simulink model "cartpole"  (R2026a)
settings: Solver=VariableStepAuto  StopTime=20
values from neighbouring files (symbols this model uses):
  Fmax = 20    [setup_cartpole.m]
  K_lqr = dlqr(Ad,Bd,Q_lqr,R_lqr)    [setup_cartpole.m]
  m = model.m    [setup_cartpole.m]
  N = numel(U)    [backward_lqr.m]    (also in forward_pass.m; ilqr.m = numel(U0); linearize_trajectory.m; setup_cartpole.m = round(T/Ts))
  s = Q*xbar          + Ak'*snext          + Ak'*Snext*Bk*d(k)    [backward_lqr.m]
  Ts = 0.01    [setup_cartpole.m]
  X = Xnew    [ilqr.m]
undefined symbols (not defined in the file or in its folder): Knom, param, Unom, Xnom, Y, Z
libraries: sm_lib x11, nesl_utility x7
settings Model: Creator=basak  LastModifiedBy=paolapinna
settings SimscapeCC: SimscapeNominalValues="[{\"value\":\"1\",\"unit\":\"A\"},{\"value\":\"1\",\"unit\":\"bar\"},{\"value\":\"1\",\"unit\":\"cm^2\"},{\"value\":\"1\",\"unit\":\"cm^3/s\"},{\"value\":\"1\",\"unit\":\"kJ/kg\"},{\"value\":\"1\",\"unit\":\"kW\"},{\"value\":\"1\",\"unit\":\"l\"},{\"value\":\"1\",\"unit\":\"N\"},{\"value\":\"1\",\"unit\":\"N*m\"},{\"value\":\"1\",\"unit\":\"V\"}]"  SimscapeLogType=none  SimscapeLogDataHistory=5000.0

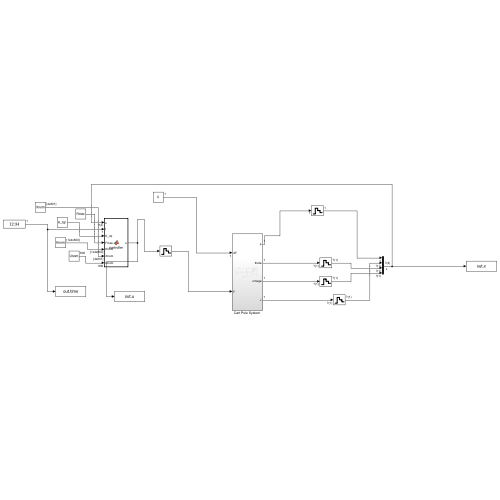
[thumbnail: Simulink's stored preview of the top-level diagram]
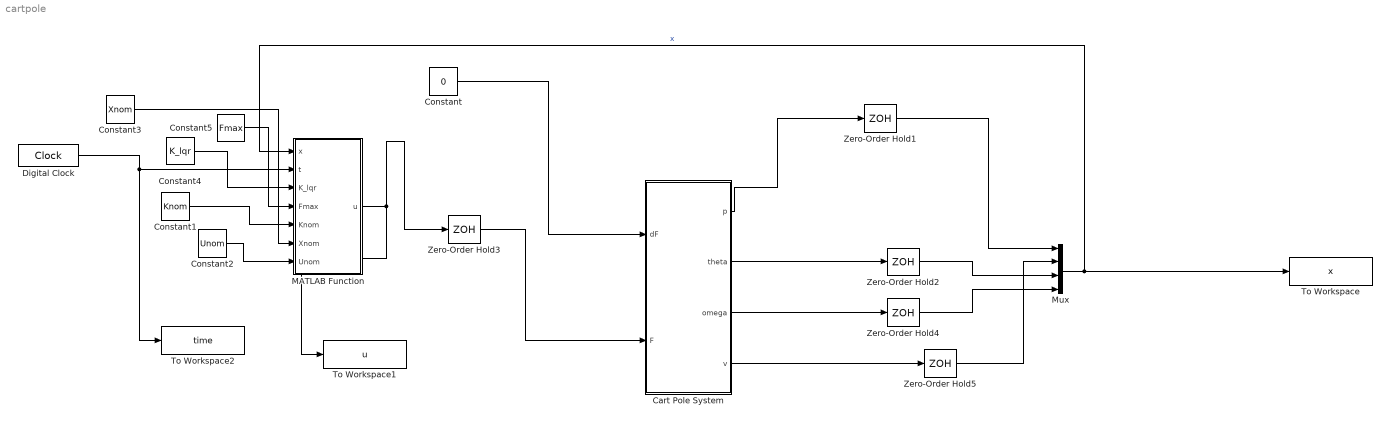
== system cartpole ==
  "Cart Pole System " : Subsystem
  Constant : Constant  Value=0
  Constant1 : Constant  Value=Knom
  Constant2 : Constant  Value=Unom
  Constant3 : Constant  Value=Xnom
  Constant4 : Constant  Value=K_lqr
  Constant5 : Constant  Value=Fmax
  Digital Clock : DigitalClock  SampleTime=Ts
  MATLAB Function : MATLAB Function  TreatAsAtomicUnit=on
  Mux : Mux
  To Workspace : ToWorkspace  VariableName=x  SaveFormat=Timeseries  SampleTime=-1
  To Workspace1 : ToWorkspace  VariableName=u  SaveFormat=Timeseries  SampleTime=-1
  To Workspace2 : ToWorkspace  VariableName=time  SaveFormat=Timeseries  SampleTime=-1
  Zero-Order Hold{1..5} (5 alike) : ZeroOrderHold  SampleTime=Ts
  wires:
  Constant/1 -> "Cart Pole System "/1(dF)
  "Cart Pole System "/1(p) -> Zero-Order Hold1/1
  "Cart Pole System "/2(theta) -> Zero-Order Hold2/1
  "Cart Pole System "/3(omega) -> Zero-Order Hold4/1
  "Cart Pole System "/4(v) -> Zero-Order Hold5/1
  MATLAB Function/1(u) -> Zero-Order Hold3/1, To Workspace1/1
  Zero-Order Hold3/1 -> "Cart Pole System "/2(F)
  Zero-Order Hold1/1 -> Mux/1
  Zero-Order Hold2/1 -> Mux/3
  Zero-Order Hold5/1 -> Mux/2
  Zero-Order Hold4/1 -> Mux/4
  Mux/1 -> To Workspace/1, MATLAB Function/1(x)  "x"
  Digital Clock/1 -> To Workspace2/1, MATLAB Function/2(t)
  Constant3/1 -> MATLAB Function/6(Xnom)
  Constant1/1 -> MATLAB Function/5(Knom)
  Constant2/1 -> MATLAB Function/7(Unom)
  Constant4/1 -> MATLAB Function/3(K_lqr)
  Constant5/1 -> MATLAB Function/4(Fmax)

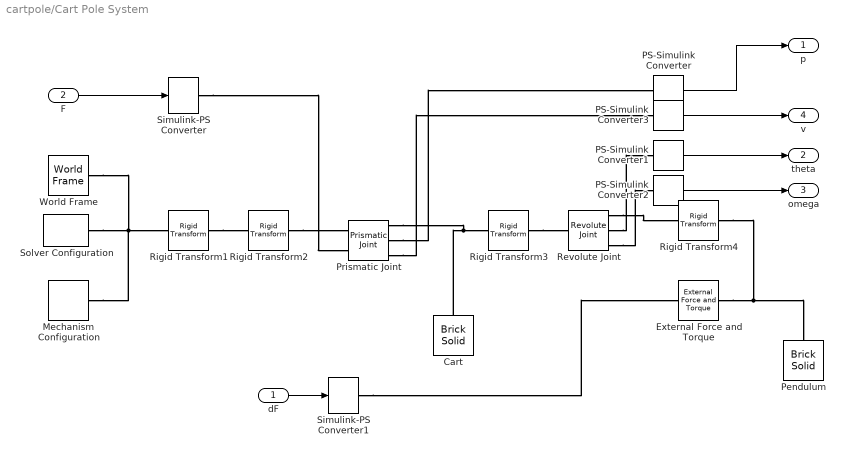
== system cartpole/Cart Pole System  ==
  dF : Inport
  F : Inport  Port=2
  Cart : sm_lib/Body Elements/Brick Solid  BrickDimensions=[param.L/6 param.L/6 param.L/3]  BrickDimensionsUnits=m  ExportEntireGeometry=off  InertiaType=PointMass  BasedOnType=Density  Density=1000  DensityUnits=kg/(m^3)  Mass=param.M  MassUnits=kg  CenterOfMass=[0 0 0]  CenterOfMassUnits=m  MomentsOfInertia=[1 1 1]  MomentsOfInertiaUnits=kg*m^2  ProductsOfInertia=[0 0 0]  ProductsOfInertiaUnits=kg*m^2  GraphicType=FromGeometry  MarkerShape=Sphere  MarkerSize=10  GraphicVisPropType=SimpleVisualProperties  GraphicDiffuseColor=[0.5 0.5 0.5]  GraphicOpacity=1.0  GraphicSpecularColor=[0.5 0.5 0.5 1.0]  GraphicAmbientColor=[0.15 0.15 0.15 1.0]  GraphicEmissiveColor=[0.0 0.0 0.0 1.0]  GraphicShininess=75  DoExposeReferenceFrame=on  SerializedFrames=<Frames/>
  External Force and Torque : sm_lib/Forces and Torques/External Force and Torque  EnableForceX=on  EnableForceY=off  EnableForceZ=off  EnableForce=off  ForceResolutionFrame=World  EnableTorqueX=off  EnableTorqueY=off  EnableTorqueZ=off  EnableTorque=off  TorqueResolutionFrame=AttachedFrame
  Mechanism Configuration : sm_lib/Utilities/Mechanism Configuration  UniformGravity=Constant  GravityVector=[0 0 -9.81]  GravityVectorUnits=m/s^2  LinearizationDelta=0.001  JointModeTransitionNonlinearIterations=2
  PS-Simulink Converter{,1..3} (4 alike) : nesl_utility/PS-Simulink Converter  PhysicalDomain=network_engine_domain  SubClassName=ps_output  LeftPortType=input  RightPortType=output  PseudoPeriodic=off  Frequencies=[]  VectorFormat=1-D array  Unit=1  AffineConversion=off
  Pendulum : sm_lib/Body Elements/Brick Solid  BrickDimensions=[param.L param.L/12 param.L/12]  BrickDimensionsUnits=m  ExportEntireGeometry=off  InertiaType=PointMass  BasedOnType=Density  Density=1000  DensityUnits=kg/(m^3)  Mass=param.m  MassUnits=kg  CenterOfMass=[0 0 0]  CenterOfMassUnits=m  MomentsOfInertia=[1 1 1]  MomentsOfInertiaUnits=kg*m^2  ProductsOfInertia=[0 0 0]  ProductsOfInertiaUnits=kg*m^2  GraphicType=FromGeometry  MarkerShape=Sphere  MarkerSize=10  GraphicVisPropType=SimpleVisualProperties  GraphicDiffuseColor=[0.8 0.0 0.2]  GraphicOpacity=1.0  GraphicSpecularColor=[0.5 0.5 0.5 1.0]  GraphicAmbientColor=[0.15 0.15 0.15 1.0]  GraphicEmissiveColor=[0.0 0.0 0.0 1.0]  GraphicShininess=75  DoExposeReferenceFrame=on  SerializedFrames=<Frames/>
  Prismatic Joint : sm_lib/Joints/Prismatic Joint  JointMode=Normal  CompositeWrenchDir=FollowerOnBase  CompositeWrenchFrame=BaseFrame  SenseConstraintForce=off  SenseConstraintTorque=off  SenseTotalForce=off  SenseTotalTorque=off  PositionTargetSpecify=on  PositionTargetPriority=High  PositionTargetValue=param.p0  PositionTargetValueUnits=m  VelocityTargetSpecify=on  VelocityTargetPriority=High  VelocityTargetValue=param.v0  VelocityTargetValueUnits=m/s  EquilibriumPosition=0  EquilibriumPositionUnits=m  SpringStiffness=0  SpringStiffnessUnits=N/m  DampingCoefficient=param.bc  DampingCoefficientUnits=N/(m/s)  LowerLimitSpecify=off  LowerLimitBound=-1  LowerLimitBoundUnits=m  LowerLimitStiffness=1e6  LowerLimitStiffnessUnits=N/m  LowerLimitDamping=1e3  LowerLimitDampingUnits=N/(m/s)  LowerLimitTransitionRegionWidth=1e-4  LowerLimitTransitionRegionWidthUnits=m  UpperLimitSpecify=off  UpperLimitBound=1  UpperLimitBoundUnits=m  UpperLimitStiffness=1e6  UpperLimitStiffnessUnits=N/m  UpperLimitDamping=1e3  UpperLimitDampingUnits=N/(m/s)  UpperLimitTransitionRegionWidth=1e-4  UpperLimitTransitionRegionWidthUnits=m  TorqueActuationMode=InputTorque  MotionActuationMode=ComputedMotion  SensePosition=on  SenseVelocity=on  SenseAcceleration=off  SenseTorqueForce=off  SenseLowerLimitTorqueForce=off  SenseUpperLimitTorqueForce=off
  Revolute Joint : sm_lib/Joints/Revolute Joint  JointMode=Normal  CompositeWrenchDir=FollowerOnBase  CompositeWrenchFrame=BaseFrame  SenseConstraintForce=off  SenseConstraintTorque=off  SenseTotalForce=off  SenseTotalTorque=off  PositionTargetSpecify=on  PositionTargetPriority=High  PositionTargetValue=param.theta0  PositionTargetValueUnits=deg  VelocityTargetSpecify=on  VelocityTargetPriority=High  VelocityTargetValue=param.omega0  VelocityTargetValueUnits=rad/s  EquilibriumPosition=0  EquilibriumPositionUnits=deg  SpringStiffness=0  SpringStiffnessUnits=N*m/deg  DampingCoefficient=param.bp  DampingCoefficientUnits=N*m/(rad/s)  LowerLimitSpecify=off  LowerLimitBound=-90  LowerLimitBoundUnits=deg  LowerLimitStiffness=1e4  LowerLimitStiffnessUnits=N*m/deg  LowerLimitDamping=10  LowerLimitDampingUnits=N*m/(deg/s)  LowerLimitTransitionRegionWidth=0.1  LowerLimitTransitionRegionWidthUnits=deg  UpperLimitSpecify=off  UpperLimitBound=90  UpperLimitBoundUnits=deg  UpperLimitStiffness=1e4  UpperLimitStiffnessUnits=N*m/deg  UpperLimitDamping=10  UpperLimitDampingUnits=N*m/(deg/s)  UpperLimitTransitionRegionWidth=0.1  UpperLimitTransitionRegionWidthUnits=deg  TorqueActuationMode=NoTorque  MotionActuationMode=ComputedMotion  SensePosition=on  SenseVelocity=on  SenseAcceleration=off  SenseTorqueForce=off  SenseLowerLimitTorqueForce=off  SenseUpperLimitTorqueForce=off
  Rigid Transform1 : sm_lib/Frames and Transforms/Rigid Transform  RotationMethod=StandardAxis  FollAlignAxisA=+X  BaseAlignAxisA=+Y  FollAlignAxisB=+Y  BaseAlignAxisB=+Z  RotationStandardAxis=+Y  RotationAngle=90  RotationAngleUnits=deg  RotationArbitraryAxis=[0 0 1]  RotationSequenceAxes=FollowerAxes  RotationSequence=XYX  RotationSequenceAngles=[0 0 0]  RotationSequenceAnglesUnits=deg  RotationMatrix=[1 0 0; 0 1 0; 0 0 1]  Quaternion=[1 0 0 0]  TranslationMethod=None  TranslationCartesianOffset=[0 0 0]  TranslationCartesianOffsetUnits=m  TranslationStandardAxis=+Z  TranslationStandardOffset=0  TranslationStandardOffsetUnits=m  TranslationROffset=0  TranslationROffsetUnits=m  TranslationThetaOffset=0  TranslationThetaOffsetUnits=deg  TranslationZOffset=0  TranslationZOffsetUnits=m
  Rigid Transform2 : sm_lib/Frames and Transforms/Rigid Transform  RotationMethod=StandardAxis  FollAlignAxisA=+X  BaseAlignAxisA=+Y  FollAlignAxisB=+Y  BaseAlignAxisB=+Z  RotationStandardAxis=+Z  RotationAngle=180  RotationAngleUnits=deg  RotationArbitraryAxis=[0 0 1]  RotationSequenceAxes=FollowerAxes  RotationSequence=XYX  RotationSequenceAngles=[0 0 0]  RotationSequenceAnglesUnits=deg  RotationMatrix=[1 0 0; 0 1 0; 0 0 1]  Quaternion=[1 0 0 0]  TranslationMethod=None  TranslationCartesianOffset=[0 0 0]  TranslationCartesianOffsetUnits=m  TranslationStandardAxis=+Z  TranslationStandardOffset=0  TranslationStandardOffsetUnits=m  TranslationROffset=0  TranslationROffsetUnits=m  TranslationThetaOffset=0  TranslationThetaOffsetUnits=deg  TranslationZOffset=0  TranslationZOffsetUnits=m
  Rigid Transform3 : sm_lib/Frames and Transforms/Rigid Transform  RotationMethod=StandardAxis  FollAlignAxisA=+X  BaseAlignAxisA=+Y  FollAlignAxisB=+Y  BaseAlignAxisB=+Z  RotationStandardAxis=-X  RotationAngle=90  RotationAngleUnits=deg  RotationArbitraryAxis=[0 0 1]  RotationSequenceAxes=FollowerAxes  RotationSequence=XYX  RotationSequenceAngles=[0 0 0]  RotationSequenceAnglesUnits=deg  RotationMatrix=[1 0 0; 0 1 0; 0 0 1]  Quaternion=[1 0 0 0]  TranslationMethod=None  TranslationCartesianOffset=[0 0 0]  TranslationCartesianOffsetUnits=m  TranslationStandardAxis=+Z  TranslationStandardOffset=0  TranslationStandardOffsetUnits=m  TranslationROffset=0  TranslationROffsetUnits=m  TranslationThetaOffset=0  TranslationThetaOffsetUnits=deg  TranslationZOffset=0  TranslationZOffsetUnits=m
  Rigid Transform4 : sm_lib/Frames and Transforms/Rigid Transform  RotationMethod=StandardAxis  FollAlignAxisA=+X  BaseAlignAxisA=+Y  FollAlignAxisB=+Y  BaseAlignAxisB=+Z  RotationStandardAxis=+X  RotationAngle=90  RotationAngleUnits=deg  RotationArbitraryAxis=[0 0 1]  RotationSequenceAxes=FollowerAxes  RotationSequence=XYX  RotationSequenceAngles=[0 0 0]  RotationSequenceAnglesUnits=deg  RotationMatrix=[1 0 0; 0 1 0; 0 0 1]  Quaternion=[1 0 0 0]  TranslationMethod=StandardAxis  TranslationCartesianOffset=[0 0 0]  TranslationCartesianOffsetUnits=m  TranslationStandardAxis=+X  TranslationStandardOffset=param.L/2  TranslationStandardOffsetUnits=m  TranslationROffset=0  TranslationROffsetUnits=m  TranslationThetaOffset=0  TranslationThetaOffsetUnits=deg  TranslationZOffset=0  TranslationZOffsetUnits=m
  Simulink-PS Converter : nesl_utility/Simulink-PS Converter  PhysicalDomain=network_engine_domain  SubClassName=ps_input  LeftPortType=input  RightPortType=output  PseudoPeriodic=off  Frequencies=[]  NoiseDistribution=none  NoiseParameters=[]  Unit=1  AffineConversion=off  FilteringAndDerivatives=zero  SimscapeFilterOrder=1  InputFilterTimeConstant=0.001  UdotUserProvided=1
  Simulink-PS Converter1 : nesl_utility/Simulink-PS Converter  PhysicalDomain=network_engine_domain  SubClassName=ps_input  LeftPortType=input  RightPortType=output  PseudoPeriodic=off  Frequencies=[]  NoiseDistribution=none  NoiseParameters=[]  Unit=1  AffineConversion=off  FilteringAndDerivatives=zero  SimscapeFilterOrder=1  InputFilterTimeConstant=0.001  UdotUserProvided=1
  Solver Configuration : nesl_utility/Solver Configuration  PhysicalDomain=network_engine_domain  SubClassName=solver  LeftPortType=input  RightPortType=generic  Tones=[]  Harmonics=[]  SimulateNoise=off  Profile=off  UseLocalSampling=off  EnableSwitchedLinearOptims=on  FrequencyDomain=off  UseCCode=off  RelTol=0.001  AbsTol=1e-06  MinStep=1e-09  ToWorkspace=off  RevertToSquareIcSolve=off  NumHomotopyIterations=100  PhasorMode=off  PhasorModeNumHarmonics=1  ConsistencySolver=NEWTON_FTOL  CanonicalOrdering=UNORDERED  OptimizeIntermediates=UNOPTIMIZED  IndexReductionMethod=DerivativeReplacement  DoDC=off  ResidualTolerance=1e-09  ConsistencyTolSource=GLOBAL  ConsistencyAbsTol=0.001  ConsistencyRelTol=0.001  ConsistencyTolFactor=0.001  UseLocalSolver=off  LocalSolverChoice=NE_BACKWARD_EULER_ADVANCER  ResolveIndetEquations=on  FunctionEvalNumThread=1  LocalSolverSampleTime=0.001  DoFixedCost=off  MaxNonlinIter=3  MaxModeIter=2  ComputeImpulses=off  ImpulseIterations=2  LinearAlgebra=Sparse  LinearAlgebraNumThread=0  EquationFormulation=NE_TIME_EF  DelaysMemoryBudget=1024  AutomaticFiltering=on  FilteringTimeConstant=0.001  PartitionStorageMethod=AS_NEEDED  PartitionMemoryBudget=1024  PartitionMethod=FAST  MultibodyUseLocalSolver=off  MultibodyLocalSolverChoice=ODE1  MultibodyLocalSolverSampleTime=0.001
  World Frame : sm_lib/Frames and Transforms/World Frame
  p : Outport  VectorParamsAs1DForOutWhenUnconnected=off
  theta : Outport  Port=2  VectorParamsAs1DForOutWhenUnconnected=off
  omega : Outport  Port=3  VectorParamsAs1DForOutWhenUnconnected=off
  v : Outport  Port=4  VectorParamsAs1DForOutWhenUnconnected=off
  wires:
  PS-Simulink Converter3/1 -> v/1
  dF/1 -> Simulink-PS Converter1/1
  PS-Simulink Converter1/1 -> theta/1
  PS-Simulink Converter/1 -> p/1
  PS-Simulink Converter2/1 -> omega/1
  F/1 -> Simulink-PS Converter/1
  connections:
  Simulink-PS Converter1/RConn1 -- External Force and Torque/LConn1
  Rigid Transform3/RConn1 -- Revolute Joint/LConn1
  Prismatic Joint/RConn3 -- PS-Simulink Converter3/LConn1
  Simulink-PS Converter/RConn1 -- Prismatic Joint/LConn2
  Prismatic Joint/RConn2 -- PS-Simulink Converter/LConn1
  Rigid Transform2/RConn1 -- Prismatic Joint/LConn1
  World Frame/RConn1 -- Mechanism Configuration/RConn1 -- Rigid Transform1/LConn1 -- Solver Configuration/RConn1
  Rigid Transform4/RConn1 -- Pendulum/RConn1 -- External Force and Torque/RConn1
  Cart/RConn1 -- Prismatic Joint/RConn1 -- Rigid Transform3/LConn1
  Rigid Transform1/RConn1 -- Rigid Transform2/LConn1
  Revolute Joint/RConn1 -- Rigid Transform4/LConn1
  Revolute Joint/RConn2 -- PS-Simulink Converter1/LConn1
  Revolute Joint/RConn3 -- PS-Simulink Converter2/LConn1

== matlab function cartpole/MATLAB Function ==
  data: x input; t input; K_lqr input; Fmax input; u output; Knom input; Xnom input; Unom input
function u = controller(x,t,K_lqr,Fmax,Knom,Xnom,Unom)

% x = [p; v; theta; omega]

%% Force state to be a column vector
x = reshape(x,4,1);

%% Force LQR gain to be a row vector
K_lqr_row = reshape(K_lqr,1,4);

%% Sampling time
Ts = 0.01;

%% Remember whether capture already occurred
persistent captured

if isempty(captured)
    captured = false;
end

% Reset at beginning of simulation
if t < Ts/2
    captured = false;
end

%% Wrap angle
theta = atan2(sin(x(3)),cos(x(3)));

%% Current state
x_current = [x(1);
             x(2);
             theta;
             x(4)];

%% Capture zone
captureBounds = [0.4;
                 0.5;
                 20*pi/180;
                 2.0];

%% Check capture condition
if ~captured && all(abs(x_current) <= captureBounds)
    captured = true;
end

%% Controller selection

if captured

    % ============================================================
    % Upright LQR
    % ============================================================
    u_raw = -K_lqr_row*x_current;

else

    % ============================================================
    % iLQR trajectory tracking
    % ============================================================

    k = floor(t/Ts + 1e-7) + 1;

    % If trajectory has finished before capture
    if k > length(Unom)
        u_raw = 0;
    else

        % Nominal state error
        dx = x_current - Xnom(:,k);

        % Shortest angular error
        dx(3) = atan2(sin(dx(3)),cos(dx(3)));

        % iLQR feedback
        Kk = reshape(Knom(:,:,k),1,4);

        u_raw = Unom(k) - Kk*dx;

    end

end

%% Force saturation
u = min(max(u_raw,-Fmax),Fmax);

end
